simulink model "Main_SpeedOptimisedVersionTannenweg"  (R2024b)
settings: Solver=ode15s  StartTime=0.0  StopTime=3600*2  FixedStep=0.1  RelTol=0.001
model workspace (MAT data in the model file):
  Ti = 5
  fa = 0.00071
  fd = 0.03
  ips = 36
  ma = 0.0013
  md = 0.04
  roomarea1 = 20
  s = 15
libraries: fl_lib x1434, nesl_utility x105, SimscapeFluids_lib x35
(part 4 of 22)

== system Main_SpeedOptimisedVersionTannenweg/EG/Raum12 ==
  Tatm : Inport
  valve command : Inport  Port=2
  Air-InnerDoor Convection1 : fl_lib/Thermal/Thermal Elements/Convective Heat Transfer  thermal_type=foundation.enum.constant_variable.constant  area=1.8 m^2  heat_tr_coeff=8 W/m^2/K  min_heat_tr_coeff=1e-3 W/(K*m^2)  T_specify=off  T_priority=High  T=0 K  T_nominal_specify=off  T_nominal_value=1  T_nominal_unit=K  Q_specify=off  Q_priority=High  Q=0 J/s  Q_nominal_specify=off  Q_nominal_value=1  Q_nominal_unit=W
  Controlled Temperature Source : fl_lib/Thermal/Thermal Sources/Controlled Temperature Source
  Flur12OG2 : fl_lib/Thermal/Thermal Elements/Convective Heat Transfer  thermal_type=foundation.enum.constant_variable.constant  area=19.68 m^2  heat_tr_coeff=8 W/m^2/K  min_heat_tr_coeff=1e-3 W/(K*m^2)  T_specify=off  T_priority=High  T=0 K  T_nominal_specify=off  T_nominal_value=1  T_nominal_unit=K  Q_specify=off  Q_priority=High  Q=0 J/s  Q_nominal_specify=off  Q_nominal_value=1  Q_nominal_unit=W
  Half Flur12OG2 : fl_lib/Thermal/Thermal Elements/Conductive Heat Transfer  thermal_type=foundation.enum.ConstantVariableTabulated.Constant  wall_geometry=foundation.enum.ConductionWallGeometry.Planar  area=19.68 m^2  thickness=.15 m  d_in=0.05 m  d_out=0.1 m  L=1 m  th_cond_min=10 W/(K*m)  th_cond=.32 W/m/K  th_cond_TLU=[413, 401, 392, 383, 371, 357, 342] W/(K*m)  temp_TLU=[200, 273, 400, 600, 800, 1000, 1200] K  T_specify=off  T_priority=High  T=0 K  T_nominal_specify=off  T_nominal_value=1  T_nominal_unit=K  Q_specify=off  Q_priority=High  Q=0 J/s  Q_nominal_specify=off  Q_nominal_value=1  Q_nominal_unit=W
  Half IW1-Air4 : fl_lib/Thermal/Thermal Elements/Conductive Heat Transfer  thermal_type=foundation.enum.ConstantVariableTabulated.Constant  wall_geometry=foundation.enum.ConductionWallGeometry.Planar  area=3.1 m^2  thickness=.16 m  d_in=0.05 m  d_out=0.1 m  L=1 m  th_cond_min=10 W/(K*m)  th_cond=.069 W/m/K  th_cond_TLU=[413, 401, 392, 383, 371, 357, 342] W/(K*m)  temp_TLU=[200, 273, 400, 600, 800, 1000, 1200] K  T_specify=off  T_priority=High  T=0 K  T_nominal_specify=off  T_nominal_value=1  T_nominal_unit=K  Q_specify=off  Q_priority=High  Q=0 J/s  Q_nominal_specify=off  Q_nominal_value=1  Q_nominal_unit=W
  Half Wall-Air Conduction1 : fl_lib/Thermal/Thermal Elements/Conductive Heat Transfer  thermal_type=foundation.enum.ConstantVariableTabulated.Constant  wall_geometry=foundation.enum.ConductionWallGeometry.Planar  area=3.7 m^2  thickness=.16 m  d_in=0.05 m  d_out=0.1 m  L=1 m  th_cond_min=10 W/(K*m)  th_cond=.069 W/m/K  th_cond_TLU=[413, 401, 392, 383, 371, 357, 342] W/(K*m)  temp_TLU=[200, 273, 400, 600, 800, 1000, 1200] K  T_specify=off  T_priority=High  T=0 K  T_nominal_specify=off  T_nominal_value=1  T_nominal_unit=K  Q_specify=off  Q_priority=High  Q=0 J/s  Q_nominal_specify=off  Q_nominal_value=1  Q_nominal_unit=W
  Half Wall-Air Conduction2 : fl_lib/Thermal/Thermal Elements/Conductive Heat Transfer  thermal_type=foundation.enum.ConstantVariableTabulated.Constant  wall_geometry=foundation.enum.ConductionWallGeometry.Planar  area=8.4 m^2  thickness=.16 m  d_in=0.05 m  d_out=0.1 m  L=1 m  th_cond_min=10 W/(K*m)  th_cond=.069 W/m/K  th_cond_TLU=[413, 401, 392, 383, 371, 357, 342] W/(K*m)  temp_TLU=[200, 273, 400, 600, 800, 1000, 1200] K  T_specify=off  T_priority=High  T=0 K  T_nominal_specify=off  T_nominal_value=1  T_nominal_unit=K  Q_specify=off  Q_priority=High  Q=0 J/s  Q_nominal_specify=off  Q_nominal_value=1  Q_nominal_unit=W
  Half Wall-Air Conduction3 : fl_lib/Thermal/Thermal Elements/Conductive Heat Transfer  thermal_type=foundation.enum.ConstantVariableTabulated.Constant  wall_geometry=foundation.enum.ConductionWallGeometry.Planar  area=12.5 m^2  thickness=.16 m  d_in=0.05 m  d_out=0.1 m  L=1 m  th_cond_min=10 W/(K*m)  th_cond=.069 W/m/K  th_cond_TLU=[413, 401, 392, 383, 371, 357, 342] W/(K*m)  temp_TLU=[200, 273, 400, 600, 800, 1000, 1200] K  T_specify=off  T_priority=High  T=0 K  T_nominal_specify=off  T_nominal_value=1  T_nominal_unit=K  Q_specify=off  Q_priority=High  Q=0 J/s  Q_nominal_specify=off  Q_nominal_value=1  Q_nominal_unit=W
  Half Window-Air Conduction1 : fl_lib/Thermal/Thermal Elements/Conductive Heat Transfer  thermal_type=foundation.enum.ConstantVariableTabulated.Constant  wall_geometry=foundation.enum.ConductionWallGeometry.Planar  area=1.8 m^2  thickness=.022 m  d_in=0.05 m  d_out=0.1 m  L=1 m  th_cond_min=10 W/(K*m)  th_cond=.13 W/m/K  th_cond_TLU=[413, 401, 392, 383, 371, 357, 342] W/(K*m)  temp_TLU=[200, 273, 400, 600, 800, 1000, 1200] K  T_specify=off  T_priority=High  T=0 K  T_nominal_specify=off  T_nominal_value=1  T_nominal_unit=K  Q_specify=off  Q_priority=High  Q=0 J/s  Q_nominal_specify=off  Q_nominal_value=1  Q_nominal_unit=W
  Heater : Subsystem
      settings: PortSchema="{\"entries\":[{\"content\":{\"sides\":[{\"content\":{\"connectorIds\":[\"In1\"]},\"type\":\"ConnectorPlacement.EquallySpacedRectSide\",\"uuid\":\"7b4379d5-fe86-4f5f-b347-17463247d5cb\"},{\"content\":{\"connectorIds\":[\"RConn1\"],\"side\":\"RIGHT\"},\"type\":\"ConnectorPlacement.EquallySpacedRectSide\",\"uuid\":\"add3919f-9a79-4726-aacf-5344366c736f\"},{\"content\":{\"connectorIds\":[\"LConn1\"],\"side\":\"TOP\"},\"type\":\"ConnectorPlacement.EquallySpacedRectSide\",\"uuid\":\"2be7b118-9114-410d-904a-4756a3068fbb\"},{\"content\":{\"connectorIds\":[\"RConn2\"],\"side\":\"BOTTOM\"},\"type\":\"ConnectorPlacement.EquallySpacedRectSide\",\"uuid\":\"3477f1e1-5c09-4719-a7a1-17d4fd79a7ad\"}]},\"type\":\"ConnectorPlacement.EquallySpacedConnector\",\"uuid\":\"01d92670-8519-469a-8463-0c3952b88216\"}],\"packageUris\":[\"http://schema.mathworks.com/mf0/Connector/R2020b\"],\"version\":\"1.0\"}"
  IW12-11 : fl_lib/Thermal/Thermal Elements/Convective Heat Transfer  thermal_type=foundation.enum.constant_variable.constant  area=12.5 m^2  heat_tr_coeff=8 W/m^2/K  min_heat_tr_coeff=1e-3 W/(K*m^2)  T_specify=off  T_priority=High  T=0 K  T_nominal_specify=off  T_nominal_value=1  T_nominal_unit=K  Q_specify=off  Q_priority=High  Q=0 J/s  Q_nominal_specify=off  Q_nominal_value=1  Q_nominal_unit=W
  IW12-2 : fl_lib/Thermal/Thermal Elements/Convective Heat Transfer  thermal_type=foundation.enum.constant_variable.constant  area=3.7 m^2  heat_tr_coeff=8 W/m^2/K  min_heat_tr_coeff=1e-3 W/(K*m^2)  T_specify=off  T_priority=High  T=0 K  T_nominal_specify=off  T_nominal_value=1  T_nominal_unit=K  Q_specify=off  Q_priority=High  Q=0 J/s  Q_nominal_specify=off  Q_nominal_value=1  Q_nominal_unit=W
  IW12-3 : fl_lib/Thermal/Thermal Elements/Convective Heat Transfer  thermal_type=foundation.enum.constant_variable.constant  area=8.4 m^2  heat_tr_coeff=8 W/m^2/K  min_heat_tr_coeff=1e-3 W/(K*m^2)  T_specify=off  T_priority=High  T=0 K  T_nominal_specify=off  T_nominal_value=1  T_nominal_unit=K  Q_specify=off  Q_priority=High  Q=0 J/s  Q_nominal_specify=off  Q_nominal_value=1  Q_nominal_unit=W
  IW5 : fl_lib/Thermal/Thermal Elements/Convective Heat Transfer  thermal_type=foundation.enum.constant_variable.constant  area=3.1 m^2  heat_tr_coeff=8 W/m^2/K  min_heat_tr_coeff=1e-3 W/(K*m^2)  T_specify=off  T_priority=High  T=0 K  T_nominal_specify=off  T_nominal_value=1  T_nominal_unit=K  Q_specify=off  Q_priority=High  Q=0 J/s  Q_nominal_specify=off  Q_nominal_value=1  Q_nominal_unit=W
  Simulink-PS Converter3 : nesl_utility/Simulink-PS Converter  PhysicalDomain=network_engine_domain  SubClassName=ps_input  LeftPortType=input  RightPortType=output  PseudoPeriodic=off  Frequencies=[]  NoiseDistribution=none  NoiseParameters=[]  Unit=degC  AffineConversion=on  FilteringAndDerivatives=zero  SimscapeFilterOrder=1  InputFilterTimeConstant=.001  UdotUserProvided=0
  Temp. Sensor : Subsystem
  Thermal Mass Air : fl_lib/Thermal/Thermal Elements/Thermal Mass  mass_type=foundation.enum.constant_variable.constant  mass=60.4 kg  sp_heat=1005 J/kg/K  mass_min=1e-6 kg  num_ports=foundation.enum.numPorts2.one  m_specify=off  m_priority=High  m=1 kg  m_nominal_specify=off  m_nominal_value=1  m_nominal_unit=kg  T_specify=on  T_priority=High  T=Ti degC  T_nominal_specify=off  T_nominal_value=1  T_nominal_unit=K  Q_specify=off  Q_priority=None  Q=0 W  Q_nominal_specify=off  Q_nominal_value=1  Q_nominal_unit=W
  Thermal Mass Flur12OG2 : fl_lib/Thermal/Thermal Elements/Thermal Mass  mass_type=foundation.enum.constant_variable.constant  mass=5547 kg  sp_heat=889 J/kg/K  mass_min=1e-6 kg  num_ports=foundation.enum.numPorts2.one  m_specify=off  m_priority=High  m=1 kg  m_nominal_specify=off  m_nominal_value=1  m_nominal_unit=kg  T_specify=on  T_priority=High  T=Ti degC  T_nominal_specify=off  T_nominal_value=1  T_nominal_unit=K  Q_specify=off  Q_priority=None  Q=0 W  Q_nominal_specify=off  Q_nominal_value=1  Q_nominal_unit=W
  Thermal Mass IW1 : fl_lib/Thermal/Thermal Elements/Thermal Mass  mass_type=foundation.enum.constant_variable.constant  mass=8.4*547*.3*.5 kg  sp_heat=876 J/kg/K  mass_min=1e-6 kg  num_ports=foundation.enum.numPorts2.one  m_specify=off  m_priority=High  m=1 kg  m_nominal_specify=off  m_nominal_value=1  m_nominal_unit=kg  T_specify=on  T_priority=High  T=Ti degC  T_nominal_specify=off  T_nominal_value=1  T_nominal_unit=K  Q_specify=off  Q_priority=None  Q=0 W  Q_nominal_specify=off  Q_nominal_value=1  Q_nominal_unit=W
  Thermal Mass IW12 : fl_lib/Thermal/Thermal Elements/Thermal Mass  mass_type=foundation.enum.constant_variable.constant  mass=3.7*547*.3*.5 kg  sp_heat=876 J/kg/K  mass_min=1e-6 kg  num_ports=foundation.enum.numPorts2.one  m_specify=off  m_priority=High  m=1 kg  m_nominal_specify=off  m_nominal_value=1  m_nominal_unit=kg  T_specify=on  T_priority=High  T=Ti degC  T_nominal_specify=off  T_nominal_value=1  T_nominal_unit=K  Q_specify=off  Q_priority=None  Q=0 W  Q_nominal_specify=off  Q_nominal_value=1  Q_nominal_unit=W
  Thermal Mass IW2 : fl_lib/Thermal/Thermal Elements/Thermal Mass  mass_type=foundation.enum.constant_variable.constant  mass=12.5*547*.3*.5 kg  sp_heat=876 J/kg/K  mass_min=1e-6 kg  num_ports=foundation.enum.numPorts2.one  m_specify=off  m_priority=High  m=1 kg  m_nominal_specify=off  m_nominal_value=1  m_nominal_unit=kg  T_specify=on  T_priority=High  T=Ti degC  T_nominal_specify=off  T_nominal_value=1  T_nominal_unit=K  Q_specify=off  Q_priority=None  Q=0 W  Q_nominal_specify=off  Q_nominal_value=1  Q_nominal_unit=W
  Thermal Mass IW5 : fl_lib/Thermal/Thermal Elements/Thermal Mass  mass_type=foundation.enum.constant_variable.constant  mass=1 kg  sp_heat=1600 J/kg/K  mass_min=1e-6 kg  num_ports=foundation.enum.numPorts2.one  m_specify=off  m_priority=High  m=1 kg  m_nominal_specify=off  m_nominal_value=1  m_nominal_unit=kg  T_specify=on  T_priority=High  T=Ti degC  T_nominal_specify=off  T_nominal_value=1  T_nominal_unit=K  Q_specify=off  Q_priority=None  Q=0 W  Q_nominal_specify=off  Q_nominal_value=1  Q_nominal_unit=W
  Thermal Mass InnerDoor : fl_lib/Thermal/Thermal Elements/Thermal Mass  mass_type=foundation.enum.constant_variable.constant  mass=36 kg  sp_heat=1600 J/kg/K  mass_min=1e-6 kg  num_ports=foundation.enum.numPorts2.one  m_specify=off  m_priority=High  m=1 kg  m_nominal_specify=off  m_nominal_value=1  m_nominal_unit=kg  T_specify=on  T_priority=High  T=Ti degC  T_nominal_specify=off  T_nominal_value=1  T_nominal_unit=K  Q_specify=off  Q_priority=None  Q=0 W  Q_nominal_specify=off  Q_nominal_value=1  Q_nominal_unit=W
  Thermal Reference1 : fl_lib/Thermal/Thermal Elements/Thermal Reference
  X-Atm : Subsystem
  Hot Water In1 : PMIOPort  Side=Left
  Hot Water Out1 : PMIOPort  Port=2  Side=Left
  Y-6 Flur12OG2 : PMIOPort  Port=3  Side=Left
  12-11 : PMIOPort  Port=4  Side=Right
  Door12 : PMIOPort  Port=5  Side=Right
  12-3 : PMIOPort  Port=6  Side=Right
  12-2 : PMIOPort  Port=7  Side=Right
  Troom : Outport
  wires:
  Tatm/1 -> Simulink-PS Converter3/1
  Temp. Sensor/1(T) -> Troom/1
  valve command/1 -> Heater/1(valve command)
  connections:
  Flur12OG2/RConn1 -- Half Flur12OG2/LConn1
  Half Flur12OG2/RConn1 -- Thermal Mass Flur12OG2/LConn1 -- Y-6 Flur12OG2/RConn1
  IW5/RConn1 -- Half IW1-Air4/LConn1
  Thermal Mass IW5/LConn1 -- Half IW1-Air4/RConn1
  Heater/RConn2 -- Hot Water Out1/RConn1
  Hot Water In1/RConn1 -- Heater/LConn1
  X-Atm/RConn1 -- Controlled Temperature Source/LConn1
  IW12-11/LConn1 -- Flur12OG2/LConn1 -- IW5/LConn1 -- Air-InnerDoor Convection1/LConn1 -- IW12-3/LConn1 -- Heater/RConn1 -- Thermal Mass Air/LConn1 -- X-Atm/LConn1 -- Temp. Sensor/LConn1 -- IW12-2/LConn1
  Controlled Temperature Source/RConn1 -- Simulink-PS Converter3/RConn1
  Thermal Reference1/LConn1 -- Controlled Temperature Source/RConn2
  12-3/RConn1 -- Thermal Mass IW1/LConn1 -- Half Wall-Air Conduction2/RConn1
  Thermal Mass InnerDoor/LConn1 -- Half Window-Air Conduction1/RConn1 -- Door12/RConn1
  Half Wall-Air Conduction3/RConn1 -- Thermal Mass IW2/LConn1 -- 12-11/RConn1
  12-2/RConn1 -- Half Wall-Air Conduction1/RConn1 -- Thermal Mass IW12/LConn1
  IW12-11/RConn1 -- Half Wall-Air Conduction3/LConn1
  Air-InnerDoor Convection1/RConn1 -- Half Window-Air Conduction1/LConn1
  IW12-2/RConn1 -- Half Wall-Air Conduction1/LConn1
  IW12-3/RConn1 -- Half Wall-Air Conduction2/LConn1

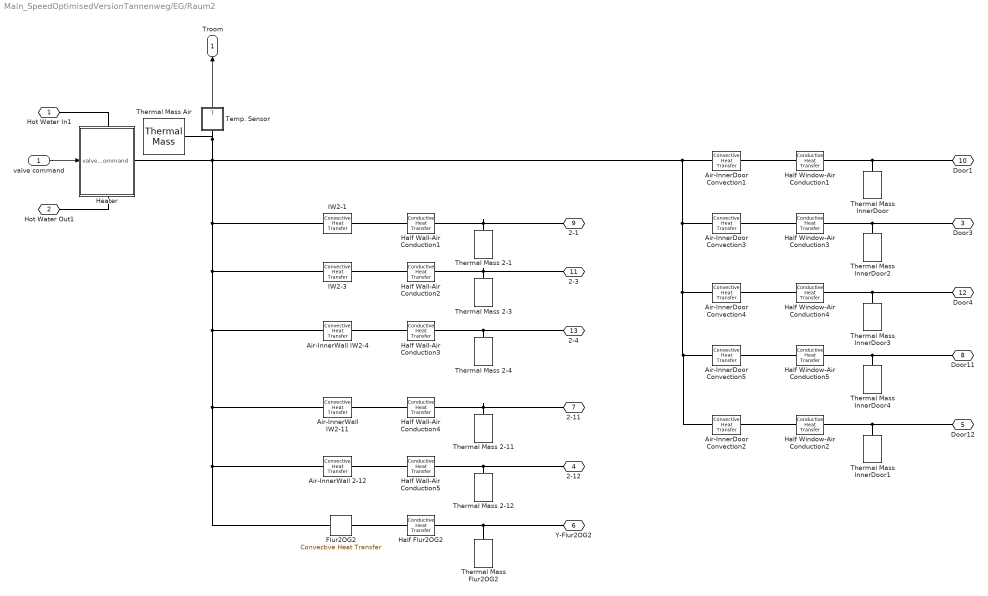
== system Main_SpeedOptimisedVersionTannenweg/EG/Raum2 ==
  valve command : Inport
  Air-InnerDoor Convection{1..5} (5 alike) : fl_lib/Thermal/Thermal Elements/Convective Heat Transfer  thermal_type=foundation.enum.constant_variable.constant  area=8.4 m^2  heat_tr_coeff=8 W/m^2/K  min_heat_tr_coeff=1e-3 W/(K*m^2)  T_specify=off  T_priority=High  T=0 K  T_nominal_specify=off  T_nominal_value=1  T_nominal_unit=K  Q_specify=off  Q_priority=High  Q=0 J/s  Q_nominal_specify=off  Q_nominal_value=1  Q_nominal_unit=W
  Air-InnerWall 2-12 : fl_lib/Thermal/Thermal Elements/Convective Heat Transfer  thermal_type=foundation.enum.constant_variable.constant  area=3.7 m^2  heat_tr_coeff=8 W/m^2/K  min_heat_tr_coeff=1e-3 W/(K*m^2)  T_specify=off  T_priority=High  T=0 K  T_nominal_specify=off  T_nominal_value=1  T_nominal_unit=K  Q_specify=off  Q_priority=High  Q=0 J/s  Q_nominal_specify=off  Q_nominal_value=1  Q_nominal_unit=W
  Air-InnerWall IW2-11 : fl_lib/Thermal/Thermal Elements/Convective Heat Transfer  thermal_type=foundation.enum.constant_variable.constant  area=1.8 m^2  heat_tr_coeff=8 W/m^2/K  min_heat_tr_coeff=1e-3 W/(K*m^2)  T_specify=off  T_priority=High  T=0 K  T_nominal_specify=off  T_nominal_value=1  T_nominal_unit=K  Q_specify=off  Q_priority=High  Q=0 J/s  Q_nominal_specify=off  Q_nominal_value=1  Q_nominal_unit=W
  Air-InnerWall IW2-4 : fl_lib/Thermal/Thermal Elements/Convective Heat Transfer  thermal_type=foundation.enum.constant_variable.constant  area=5.2 m^2  heat_tr_coeff=8 W/m^2/K  min_heat_tr_coeff=1e-3 W/(K*m^2)  T_specify=off  T_priority=High  T=0 K  T_nominal_specify=off  T_nominal_value=1  T_nominal_unit=K  Q_specify=off  Q_priority=High  Q=0 J/s  Q_nominal_specify=off  Q_nominal_value=1  Q_nominal_unit=W
  Flur2OG2 : fl_lib/Thermal/Thermal Elements/Convective Heat Transfer  thermal_type=foundation.enum.constant_variable.constant  area=5.33 m^2  heat_tr_coeff=8 W/m^2/K  min_heat_tr_coeff=1e-3 W/(K*m^2)  T_specify=off  T_priority=High  T=0 K  T_nominal_specify=off  T_nominal_value=1  T_nominal_unit=K  Q_specify=off  Q_priority=High  Q=0 J/s  Q_nominal_specify=off  Q_nominal_value=1  Q_nominal_unit=W
  Half Flur2OG2 : fl_lib/Thermal/Thermal Elements/Conductive Heat Transfer  thermal_type=foundation.enum.ConstantVariableTabulated.Constant  wall_geometry=foundation.enum.ConductionWallGeometry.Planar  area=5.33 m^2  thickness=.15 m  d_in=0.05 m  d_out=0.1 m  L=1 m  th_cond_min=10 W/(K*m)  th_cond=.32 W/m/K  th_cond_TLU=[413, 401, 392, 383, 371, 357, 342] W/(K*m)  temp_TLU=[200, 273, 400, 600, 800, 1000, 1200] K  T_specify=off  T_priority=High  T=0 K  T_nominal_specify=off  T_nominal_value=1  T_nominal_unit=K  Q_specify=off  Q_priority=High  Q=0 J/s  Q_nominal_specify=off  Q_nominal_value=1  Q_nominal_unit=W
  Half Wall-Air Conduction1 : fl_lib/Thermal/Thermal Elements/Conductive Heat Transfer  thermal_type=foundation.enum.ConstantVariableTabulated.Constant  wall_geometry=foundation.enum.ConductionWallGeometry.Planar  area=3.8 m^2  thickness=.16 m  d_in=0.05 m  d_out=0.1 m  L=1 m  th_cond_min=10 W/(K*m)  th_cond=.069 W/m/K  th_cond_TLU=[413, 401, 392, 383, 371, 357, 342] W/(K*m)  temp_TLU=[200, 273, 400, 600, 800, 1000, 1200] K  T_specify=off  T_priority=High  T=0 K  T_nominal_specify=off  T_nominal_value=1  T_nominal_unit=K  Q_specify=off  Q_priority=High  Q=0 J/s  Q_nominal_specify=off  Q_nominal_value=1  Q_nominal_unit=W
  Half Wall-Air Conduction2 : fl_lib/Thermal/Thermal Elements/Conductive Heat Transfer  thermal_type=foundation.enum.ConstantVariableTabulated.Constant  wall_geometry=foundation.enum.ConductionWallGeometry.Planar  area=6.7 m^2  thickness=.16 m  d_in=0.05 m  d_out=0.1 m  L=1 m  th_cond_min=10 W/(K*m)  th_cond=.069 W/m/K  th_cond_TLU=[413, 401, 392, 383, 371, 357, 342] W/(K*m)  temp_TLU=[200, 273, 400, 600, 800, 1000, 1200] K  T_specify=off  T_priority=High  T=0 K  T_nominal_specify=off  T_nominal_value=1  T_nominal_unit=K  Q_specify=off  Q_priority=High  Q=0 J/s  Q_nominal_specify=off  Q_nominal_value=1  Q_nominal_unit=W
  Half Wall-Air Conduction3 : fl_lib/Thermal/Thermal Elements/Conductive Heat Transfer  thermal_type=foundation.enum.ConstantVariableTabulated.Constant  wall_geometry=foundation.enum.ConductionWallGeometry.Planar  area=5.2 m^2  thickness=.16 m  d_in=0.05 m  d_out=0.1 m  L=1 m  th_cond_min=10 W/(K*m)  th_cond=.069 W/m/K  th_cond_TLU=[413, 401, 392, 383, 371, 357, 342] W/(K*m)  temp_TLU=[200, 273, 400, 600, 800, 1000, 1200] K  T_specify=off  T_priority=High  T=0 K  T_nominal_specify=off  T_nominal_value=1  T_nominal_unit=K  Q_specify=off  Q_priority=High  Q=0 J/s  Q_nominal_specify=off  Q_nominal_value=1  Q_nominal_unit=W
  Half Wall-Air Conduction4 : fl_lib/Thermal/Thermal Elements/Conductive Heat Transfer  thermal_type=foundation.enum.ConstantVariableTabulated.Constant  wall_geometry=foundation.enum.ConductionWallGeometry.Planar  area=1.8 m^2  thickness=.16 m  d_in=0.05 m  d_out=0.1 m  L=1 m  th_cond_min=10 W/(K*m)  th_cond=.069 W/m/K  th_cond_TLU=[413, 401, 392, 383, 371, 357, 342] W/(K*m)  temp_TLU=[200, 273, 400, 600, 800, 1000, 1200] K  T_specify=off  T_priority=High  T=0 K  T_nominal_specify=off  T_nominal_value=1  T_nominal_unit=K  Q_specify=off  Q_priority=High  Q=0 J/s  Q_nominal_specify=off  Q_nominal_value=1  Q_nominal_unit=W
  Half Wall-Air Conduction5 : fl_lib/Thermal/Thermal Elements/Conductive Heat Transfer  thermal_type=foundation.enum.ConstantVariableTabulated.Constant  wall_geometry=foundation.enum.ConductionWallGeometry.Planar  area=3.7 m^2  thickness=.16 m  d_in=0.05 m  d_out=0.1 m  L=1 m  th_cond_min=10 W/(K*m)  th_cond=.069 W/m/K  th_cond_TLU=[413, 401, 392, 383, 371, 357, 342] W/(K*m)  temp_TLU=[200, 273, 400, 600, 800, 1000, 1200] K  T_specify=off  T_priority=High  T=0 K  T_nominal_specify=off  T_nominal_value=1  T_nominal_unit=K  Q_specify=off  Q_priority=High  Q=0 J/s  Q_nominal_specify=off  Q_nominal_value=1  Q_nominal_unit=W
  Half Window-Air Conduction{1..5} (5 alike) : fl_lib/Thermal/Thermal Elements/Conductive Heat Transfer  thermal_type=foundation.enum.ConstantVariableTabulated.Constant  wall_geometry=foundation.enum.ConductionWallGeometry.Planar  area=8.4 m^2  thickness=.022 m  d_in=0.05 m  d_out=0.1 m  L=1 m  th_cond_min=10 W/(K*m)  th_cond=.13 W/m/K  th_cond_TLU=[413, 401, 392, 383, 371, 357, 342] W/(K*m)  temp_TLU=[200, 273, 400, 600, 800, 1000, 1200] K  T_specify=off  T_priority=High  T=0 K  T_nominal_specify=off  T_nominal_value=1  T_nominal_unit=K  Q_specify=off  Q_priority=High  Q=0 J/s  Q_nominal_specify=off  Q_nominal_value=1  Q_nominal_unit=W
  Heater : Subsystem
      settings: PortSchema="{\"entries\":[{\"content\":{\"sides\":[{\"content\":{\"connectorIds\":[\"In1\"]},\"type\":\"ConnectorPlacement.EquallySpacedRectSide\",\"uuid\":\"7b4379d5-fe86-4f5f-b347-17463247d5cb\"},{\"content\":{\"connectorIds\":[\"RConn1\"],\"side\":\"RIGHT\"},\"type\":\"ConnectorPlacement.EquallySpacedRectSide\",\"uuid\":\"add3919f-9a79-4726-aacf-5344366c736f\"},{\"content\":{\"connectorIds\":[\"LConn1\"],\"side\":\"TOP\"},\"type\":\"ConnectorPlacement.EquallySpacedRectSide\",\"uuid\":\"2be7b118-9114-410d-904a-4756a3068fbb\"},{\"content\":{\"connectorIds\":[\"RConn2\"],\"side\":\"BOTTOM\"},\"type\":\"ConnectorPlacement.EquallySpacedRectSide\",\"uuid\":\"3477f1e1-5c09-4719-a7a1-17d4fd79a7ad\"}]},\"type\":\"ConnectorPlacement.EquallySpacedConnector\",\"uuid\":\"01d92670-8519-469a-8463-0c3952b88216\"}],\"packageUris\":[\"http://schema.mathworks.com/mf0/Connector/R2020b\"],\"version\":\"1.0\"}"
  IW2-1 : fl_lib/Thermal/Thermal Elements/Convective Heat Transfer  thermal_type=foundation.enum.constant_variable.constant  area=3.8 m^2  heat_tr_coeff=8 W/m^2/K  min_heat_tr_coeff=1e-3 W/(K*m^2)  T_specify=off  T_priority=High  T=0 K  T_nominal_specify=off  T_nominal_value=1  T_nominal_unit=K  Q_specify=off  Q_priority=High  Q=0 J/s  Q_nominal_specify=off  Q_nominal_value=1  Q_nominal_unit=W
  IW2-3 : fl_lib/Thermal/Thermal Elements/Convective Heat Transfer  thermal_type=foundation.enum.constant_variable.constant  area=6.7 m^2  heat_tr_coeff=8 W/m^2/K  min_heat_tr_coeff=1e-3 W/(K*m^2)  T_specify=off  T_priority=High  T=0 K  T_nominal_specify=off  T_nominal_value=1  T_nominal_unit=K  Q_specify=off  Q_priority=High  Q=0 J/s  Q_nominal_specify=off  Q_nominal_value=1  Q_nominal_unit=W
  Temp. Sensor : Subsystem
  Thermal Mass 2-1 : fl_lib/Thermal/Thermal Elements/Thermal Mass  mass_type=foundation.enum.constant_variable.constant  mass=547*.5*.3*3.8 kg  sp_heat=876 J/kg/K  mass_min=1e-6 kg  num_ports=foundation.enum.numPorts2.one  m_specify=off  m_priority=High  m=1 kg  m_nominal_specify=off  m_nominal_value=1  m_nominal_unit=kg  T_specify=on  T_priority=High  T=Ti degC  T_nominal_specify=off  T_nominal_value=1  T_nominal_unit=K  Q_specify=off  Q_priority=None  Q=0 W  Q_nominal_specify=off  Q_nominal_value=1  Q_nominal_unit=W
  Thermal Mass 2-11 : fl_lib/Thermal/Thermal Elements/Thermal Mass  mass_type=foundation.enum.constant_variable.constant  mass=1.8*547*.15 kg  sp_heat=876 J/kg/K  mass_min=1e-6 kg  num_ports=foundation.enum.numPorts2.one  m_specify=off  m_priority=High  m=1 kg  m_nominal_specify=off  m_nominal_value=1  m_nominal_unit=kg  T_specify=on  T_priority=High  T=Ti degC  T_nominal_specify=off  T_nominal_value=1  T_nominal_unit=K  Q_specify=off  Q_priority=None  Q=0 W  Q_nominal_specify=off  Q_nominal_value=1  Q_nominal_unit=W
  Thermal Mass 2-12 : fl_lib/Thermal/Thermal Elements/Thermal Mass  mass_type=foundation.enum.constant_variable.constant  mass=3.7*547*.15 kg  sp_heat=876 J/kg/K  mass_min=1e-6 kg  num_ports=foundation.enum.numPorts2.one  m_specify=off  m_priority=High  m=1 kg  m_nominal_specify=off  m_nominal_value=1  m_nominal_unit=kg  T_specify=on  T_priority=High  T=Ti degC  T_nominal_specify=off  T_nominal_value=1  T_nominal_unit=K  Q_specify=off  Q_priority=None  Q=0 W  Q_nominal_specify=off  Q_nominal_value=1  Q_nominal_unit=W
  Thermal Mass 2-3 : fl_lib/Thermal/Thermal Elements/Thermal Mass  mass_type=foundation.enum.constant_variable.constant  mass=6.7*.15*547 kg  sp_heat=876 J/kg/K  mass_min=1e-6 kg  num_ports=foundation.enum.numPorts2.one  m_specify=off  m_priority=High  m=1 kg  m_nominal_specify=off  m_nominal_value=1  m_nominal_unit=kg  T_specify=on  T_priority=High  T=Ti degC  T_nominal_specify=off  T_nominal_value=1  T_nominal_unit=K  Q_specify=off  Q_priority=None  Q=0 W  Q_nominal_specify=off  Q_nominal_value=1  Q_nominal_unit=W
  Thermal Mass 2-4 : fl_lib/Thermal/Thermal Elements/Thermal Mass  mass_type=foundation.enum.constant_variable.constant  mass=547*.15*5.2 kg  sp_heat=876 J/kg/K  mass_min=1e-6 kg  num_ports=foundation.enum.numPorts2.one  m_specify=off  m_priority=High  m=1 kg  m_nominal_specify=off  m_nominal_value=1  m_nominal_unit=kg  T_specify=on  T_priority=High  T=Ti degC  T_nominal_specify=off  T_nominal_value=1  T_nominal_unit=K  Q_specify=off  Q_priority=None  Q=0 W  Q_nominal_specify=off  Q_nominal_value=1  Q_nominal_unit=W
  Thermal Mass Air : fl_lib/Thermal/Thermal Elements/Thermal Mass  mass_type=foundation.enum.constant_variable.constant  mass=16.4 kg  sp_heat=1005 J/kg/K  mass_min=1e-6 kg  num_ports=foundation.enum.numPorts2.one  m_specify=off  m_priority=High  m=1 kg  m_nominal_specify=off  m_nominal_value=1  m_nominal_unit=kg  T_specify=on  T_priority=High  T=Ti degC  T_nominal_specify=off  T_nominal_value=1  T_nominal_unit=K  Q_specify=off  Q_priority=None  Q=0 W  Q_nominal_specify=off  Q_nominal_value=1  Q_nominal_unit=W
  Thermal Mass Flur2OG2 : fl_lib/Thermal/Thermal Elements/Thermal Mass  mass_type=foundation.enum.constant_variable.constant  mass=1502 kg  sp_heat=889 J/kg/K  mass_min=1e-6 kg  num_ports=foundation.enum.numPorts2.one  m_specify=off  m_priority=High  m=1 kg  m_nominal_specify=off  m_nominal_value=1  m_nominal_unit=kg  T_specify=on  T_priority=High  T=Ti degC  T_nominal_specify=off  T_nominal_value=1  T_nominal_unit=K  Q_specify=off  Q_priority=None  Q=0 W  Q_nominal_specify=off  Q_nominal_value=1  Q_nominal_unit=W
  Thermal Mass InnerDoor{,1..4} (5 alike) : fl_lib/Thermal/Thermal Elements/Thermal Mass  mass_type=foundation.enum.constant_variable.constant  mass=170 kg  sp_heat=1600 J/kg/K  mass_min=1e-6 kg  num_ports=foundation.enum.numPorts2.one  m_specify=off  m_priority=High  m=1 kg  m_nominal_specify=off  m_nominal_value=1  m_nominal_unit=kg  T_specify=on  T_priority=High  T=Ti degC  T_nominal_specify=off  T_nominal_value=1  T_nominal_unit=K  Q_specify=off  Q_priority=None  Q=0 W  Q_nominal_specify=off  Q_nominal_value=1  Q_nominal_unit=W
  Hot Water In1 : PMIOPort  Side=Left
  Hot Water Out1 : PMIOPort  Port=2  Side=Left
  Door3 : PMIOPort  Port=3  Side=Left
  2-12 : PMIOPort  Port=4  Side=Left
  Door12 : PMIOPort  Port=5  Side=Left
  Y-Flur2OG2 : PMIOPort  Port=6  Side=Left
  2-11 : PMIOPort  Port=7  Side=Right
  Door11 : PMIOPort  Port=8  Side=Right
  2-1 : PMIOPort  Port=9  Side=Right
  Door1 : PMIOPort  Port=10  Side=Right
  2-3 : PMIOPort  Port=11  Side=Right
  Door4 : PMIOPort  Port=12  Side=Right
  2-4 : PMIOPort  Port=13  Side=Right
  Troom : Outport
  wires:
  Temp. Sensor/1(T) -> Troom/1
  valve command/1 -> Heater/1(valve command)
  connections:
  Heater/RConn2 -- Hot Water Out1/RConn1
  Hot Water In1/RConn1 -- Heater/LConn1
  Air-InnerWall IW2-11/LConn1 -- IW2-3/LConn1 -- IW2-1/LConn1 -- Air-InnerDoor Convection5/LConn1 -- Air-InnerDoor Convection2/LConn1 -- Air-InnerDoor Convection4/LConn1 -- Air-InnerDoor Convection3/LConn1 -- Air-InnerDoor Convection1/LConn1 -- Heater/RConn1 -- Thermal Mass Air/LConn1 -- Temp. Sensor/LConn1 -- Air-InnerWall IW2-4/LConn1 -- Flur2OG2/LConn1 -- Air-InnerWall 2-12/LConn1
  Half Window-Air Conduction3/RConn1 -- Door3/RConn1 -- Thermal Mass InnerDoor2/LConn1
  Thermal Mass 2-1/LConn1 -- Half Wall-Air Conduction1/RConn1 -- 2-1/RConn1
  Thermal Mass 2-3/LConn1 -- 2-3/RConn1 -- Half Wall-Air Conduction2/RConn1
  Thermal Mass InnerDoor3/LConn1 -- Door4/RConn1 -- Half Window-Air Conduction4/RConn1
  Thermal Mass 2-11/LConn1 -- 2-11/RConn1 -- Half Wall-Air Conduction4/RConn1
  Half Window-Air Conduction5/RConn1 -- Door11/RConn1 -- Thermal Mass InnerDoor4/LConn1
  Half Wall-Air Conduction5/RConn1 -- 2-12/RConn1 -- Thermal Mass 2-12/LConn1
  Thermal Mass InnerDoor/LConn1 -- Half Window-Air Conduction1/RConn1 -- Door1/RConn1
  Thermal Mass InnerDoor1/LConn1 -- Door12/RConn1 -- Half Window-Air Conduction2/RConn1
  Half Wall-Air Conduction3/RConn1 -- 2-4/RConn1 -- Thermal Mass 2-4/LConn1
  Air-InnerWall IW2-4/RConn1 -- Half Wall-Air Conduction3/LConn1
  Air-InnerDoor Convection2/RConn1 -- Half Window-Air Conduction2/LConn1
  Air-InnerDoor Convection4/RConn1 -- Half Window-Air Conduction4/LConn1
  Air-InnerDoor Convection1/RConn1 -- Half Window-Air Conduction1/LConn1
  Air-InnerDoor Convection3/RConn1 -- Half Window-Air Conduction3/LConn1
  IW2-3/RConn1 -- Half Wall-Air Conduction2/LConn1
  Air-InnerDoor Convection5/RConn1 -- Half Window-Air Conduction5/LConn1
  IW2-1/RConn1 -- Half Wall-Air Conduction1/LConn1
  Air-InnerWall 2-12/RConn1 -- Half Wall-Air Conduction5/LConn1
  Air-InnerWall IW2-11/RConn1 -- Half Wall-Air Conduction4/LConn1
  Thermal Mass Flur2OG2/LConn1 -- Y-Flur2OG2/RConn1 -- Half Flur2OG2/RConn1
  Flur2OG2/RConn1 -- Half Flur2OG2/LConn1

== system Main_SpeedOptimisedVersionTannenweg/EG/Raum3 ==
  Tatm : Inport
  valve command : Inport  Port=2
  Controlled Temperature Source : fl_lib/Thermal/Thermal Sources/Controlled Temperature Source
  Flur3OG2 : fl_lib/Thermal/Thermal Elements/Convective Heat Transfer  thermal_type=foundation.enum.constant_variable.constant  area=15.87 m^2  heat_tr_coeff=8 W/m^2/K  min_heat_tr_coeff=1e-3 W/(K*m^2)  T_specify=off  T_priority=High  T=0 K  T_nominal_specify=off  T_nominal_value=1  T_nominal_unit=K  Q_specify=off  Q_priority=High  Q=0 J/s  Q_nominal_specify=off  Q_nominal_value=1  Q_nominal_unit=W
  Half Flur3OG2 : fl_lib/Thermal/Thermal Elements/Conductive Heat Transfer  thermal_type=foundation.enum.ConstantVariableTabulated.Constant  wall_geometry=foundation.enum.ConductionWallGeometry.Planar  area=15.87 m^2  thickness=.15 m  d_in=0.05 m  d_out=0.1 m  L=1 m  th_cond_min=10 W/(K*m)  th_cond=.32 W/m/K  th_cond_TLU=[413, 401, 392, 383, 371, 357, 342] W/(K*m)  temp_TLU=[200, 273, 400, 600, 800, 1000, 1200] K  T_specify=off  T_priority=High  T=0 K  T_nominal_specify=off  T_nominal_value=1  T_nominal_unit=K  Q_specify=off  Q_priority=High  Q=0 J/s  Q_nominal_specify=off  Q_nominal_value=1  Q_nominal_unit=W
  Half IT-Air1 : fl_lib/Thermal/Thermal Elements/Conductive Heat Transfer  thermal_type=foundation.enum.ConstantVariableTabulated.Constant  wall_geometry=foundation.enum.ConductionWallGeometry.Planar  area=1.8 m^2  thickness=.022 m  d_in=0.05 m  d_out=0.1 m  L=1 m  th_cond_min=10 W/(K*m)  th_cond=.13 W/m/K  th_cond_TLU=[413, 401, 392, 383, 371, 357, 342] W/(K*m)  temp_TLU=[200, 273, 400, 600, 800, 1000, 1200] K  T_specify=off  T_priority=High  T=0 K  T_nominal_specify=off  T_nominal_value=1  T_nominal_unit=K  Q_specify=off  Q_priority=High  Q=0 J/s  Q_nominal_specify=off  Q_nominal_value=1  Q_nominal_unit=W
  Half IT-Air2 : fl_lib/Thermal/Thermal Elements/Conductive Heat Transfer  thermal_type=foundation.enum.ConstantVariableTabulated.Constant  wall_geometry=foundation.enum.ConductionWallGeometry.Planar  area=8.4 m^2  thickness=.022 m  d_in=0.05 m  d_out=0.1 m  L=1 m  th_cond_min=10 W/(K*m)  th_cond=.13 W/m/K  th_cond_TLU=[413, 401, 392, 383, 371, 357, 342] W/(K*m)  temp_TLU=[200, 273, 400, 600, 800, 1000, 1200] K  T_specify=off  T_priority=High  T=0 K  T_nominal_specify=off  T_nominal_value=1  T_nominal_unit=K  Q_specify=off  Q_priority=High  Q=0 J/s  Q_nominal_specify=off  Q_nominal_value=1  Q_nominal_unit=W
  Half IW1-Air : fl_lib/Thermal/Thermal Elements/Conductive Heat Transfer  thermal_type=foundation.enum.ConstantVariableTabulated.Constant  wall_geometry=foundation.enum.ConductionWallGeometry.Planar  area=6.7 m^2  thickness=.16 m  d_in=0.05 m  d_out=0.1 m  L=1 m  th_cond_min=10 W/(K*m)  th_cond=.069 W/m/K  th_cond_TLU=[413, 401, 392, 383, 371, 357, 342] W/(K*m)  temp_TLU=[200, 273, 400, 600, 800, 1000, 1200] K  T_specify=off  T_priority=High  T=0 K  T_nominal_specify=off  T_nominal_value=1  T_nominal_unit=K  Q_specify=off  Q_priority=High  Q=0 J/s  Q_nominal_specify=off  Q_nominal_value=1  Q_nominal_unit=W
  Half IW1-Air1 : fl_lib/Thermal/Thermal Elements/Conductive Heat Transfer  thermal_type=foundation.enum.ConstantVariableTabulated.Constant  wall_geometry=foundation.enum.ConductionWallGeometry.Planar  area=8.5 m^2  thickness=.16 m  d_in=0.05 m  d_out=0.1 m  L=1 m  th_cond_min=10 W/(K*m)  th_cond=.069 W/m/K  th_cond_TLU=[413, 401, 392, 383, 371, 357, 342] W/(K*m)  temp_TLU=[200, 273, 400, 600, 800, 1000, 1200] K  T_specify=off  T_priority=High  T=0 K  T_nominal_specify=off  T_nominal_value=1  T_nominal_unit=K  Q_specify=off  Q_priority=High  Q=0 J/s  Q_nominal_specify=off  Q_nominal_value=1  Q_nominal_unit=W
  Heater : Subsystem
      settings: PortSchema="{\"entries\":[{\"content\":{\"sides\":[{\"content\":{\"connectorIds\":[\"In1\"]},\"type\":\"ConnectorPlacement.EquallySpacedRectSide\",\"uuid\":\"7b4379d5-fe86-4f5f-b347-17463247d5cb\"},{\"content\":{\"connectorIds\":[\"RConn1\"],\"side\":\"RIGHT\"},\"type\":\"ConnectorPlacement.EquallySpacedRectSide\",\"uuid\":\"add3919f-9a79-4726-aacf-5344366c736f\"},{\"content\":{\"connectorIds\":[\"LConn1\"],\"side\":\"TOP\"},\"type\":\"ConnectorPlacement.EquallySpacedRectSide\",\"uuid\":\"2be7b118-9114-410d-904a-4756a3068fbb\"},{\"content\":{\"connectorIds\":[\"RConn2\"],\"side\":\"BOTTOM\"},\"type\":\"ConnectorPlacement.EquallySpacedRectSide\",\"uuid\":\"3477f1e1-5c09-4719-a7a1-17d4fd79a7ad\"}]},\"type\":\"ConnectorPlacement.EquallySpacedConnector\",\"uuid\":\"01d92670-8519-469a-8463-0c3952b88216\"}],\"packageUris\":[\"http://schema.mathworks.com/mf0/Connector/R2020b\"],\"version\":\"1.0\"}"
  IT3 : fl_lib/Thermal/Thermal Elements/Convective Heat Transfer  thermal_type=foundation.enum.constant_variable.constant  area=1.8 m^2  heat_tr_coeff=8 W/m^2/K  min_heat_tr_coeff=1e-3 W/(K*m^2)  T_specify=off  T_priority=High  T=0 K  T_nominal_specify=off  T_nominal_value=1  T_nominal_unit=K  Q_specify=off  Q_priority=High  Q=0 J/s  Q_nominal_specify=off  Q_nominal_value=1  Q_nominal_unit=W
  IW3-12 : fl_lib/Thermal/Thermal Elements/Convective Heat Transfer  thermal_type=foundation.enum.constant_variable.constant  area=8.4 m^2  heat_tr_coeff=8 W/m^2/K  min_heat_tr_coeff=1e-3 W/(K*m^2)  T_specify=off  T_priority=High  T=0 K  T_nominal_specify=off  T_nominal_value=1  T_nominal_unit=K  Q_specify=off  Q_priority=High  Q=0 J/s  Q_nominal_specify=off  Q_nominal_value=1  Q_nominal_unit=W
  IW3-2 : fl_lib/Thermal/Thermal Elements/Convective Heat Transfer  thermal_type=foundation.enum.constant_variable.constant  area=6.7 m^2  heat_tr_coeff=8 W/m^2/K  min_heat_tr_coeff=1e-3 W/(K*m^2)  T_specify=off  T_priority=High  T=0 K  T_nominal_specify=off  T_nominal_value=1  T_nominal_unit=K  Q_specify=off  Q_priority=High  Q=0 J/s  Q_nominal_specify=off  Q_nominal_value=1  Q_nominal_unit=W
  IW3-4 : fl_lib/Thermal/Thermal Elements/Convective Heat Transfer  thermal_type=foundation.enum.constant_variable.constant  area=8.5 m^2  heat_tr_coeff=8 W/m^2/K  min_heat_tr_coeff=1e-3 W/(K*m^2)  T_specify=off  T_priority=High  T=0 K  T_nominal_specify=off  T_nominal_value=1  T_nominal_unit=K  Q_specify=off  Q_priority=High  Q=0 J/s  Q_nominal_specify=off  Q_nominal_value=1  Q_nominal_unit=W
  Simulink-PS Converter3 : nesl_utility/Simulink-PS Converter  PhysicalDomain=network_engine_domain  SubClassName=ps_input  LeftPortType=input  RightPortType=output  PseudoPeriodic=off  Frequencies=[]  NoiseDistribution=none  NoiseParameters=[]  Unit=degC  AffineConversion=on  FilteringAndDerivatives=zero  SimscapeFilterOrder=1  InputFilterTimeConstant=.001  UdotUserProvided=0
  Temp. Sensor : Subsystem
  Thermal Mass 3-12 : fl_lib/Thermal/Thermal Elements/Thermal Mass  mass_type=foundation.enum.constant_variable.constant  mass=8.4*.15*547 kg  sp_heat=1600 J/kg/K  mass_min=1e-6 kg  num_ports=foundation.enum.numPorts2.one  m_specify=off  m_priority=High  m=1 kg  m_nominal_specify=off  m_nominal_value=1  m_nominal_unit=kg  T_specify=on  T_priority=High  T=Ti degC  T_nominal_specify=off  T_nominal_value=1  T_nominal_unit=K  Q_specify=off  Q_priority=None  Q=0 W  Q_nominal_specify=off  Q_nominal_value=1  Q_nominal_unit=W
  Thermal Mass Air : fl_lib/Thermal/Thermal Elements/Thermal Mass  mass_type=foundation.enum.constant_variable.constant  mass=48.7 kg  sp_heat=1005 J/kg/K  mass_min=1e-6 kg  num_ports=foundation.enum.numPorts2.one  m_specify=off  m_priority=High  m=1 kg  m_nominal_specify=off  m_nominal_value=1  m_nominal_unit=kg  T_specify=on  T_priority=High  T=Ti degC  T_nominal_specify=off  T_nominal_value=1  T_nominal_unit=K  Q_specify=off  Q_priority=None  Q=0 W  Q_nominal_specify=off  Q_nominal_value=1  Q_nominal_unit=W
  Thermal Mass Door3 : fl_lib/Thermal/Thermal Elements/Thermal Mass  mass_type=foundation.enum.constant_variable.constant  mass=36 kg  sp_heat=1600 J/kg/K  mass_min=1e-6 kg  num_ports=foundation.enum.numPorts2.one  m_specify=off  m_priority=High  m=1 kg  m_nominal_specify=off  m_nominal_value=1  m_nominal_unit=kg  T_specify=on  T_priority=High  T=Ti degC  T_nominal_specify=off  T_nominal_value=1  T_nominal_unit=K  Q_specify=off  Q_priority=None  Q=0 W  Q_nominal_specify=off  Q_nominal_value=1  Q_nominal_unit=W
  Thermal Mass Flur3OG2 : fl_lib/Thermal/Thermal Elements/Thermal Mass  mass_type=foundation.enum.constant_variable.constant  mass=4473 kg  sp_heat=889 J/kg/K  mass_min=1e-6 kg  num_ports=foundation.enum.numPorts2.one  m_specify=off  m_priority=High  m=1 kg  m_nominal_specify=off  m_nominal_value=1  m_nominal_unit=kg  T_specify=on  T_priority=High  T=Ti degC  T_nominal_specify=off  T_nominal_value=1  T_nominal_unit=K  Q_specify=off  Q_priority=None  Q=0 W  Q_nominal_specify=off  Q_nominal_value=1  Q_nominal_unit=W
  Thermal Mass IW3-2 : fl_lib/Thermal/Thermal Elements/Thermal Mass  mass_type=foundation.enum.constant_variable.constant  mass=6.7*.15*547 kg  sp_heat=1600 J/kg/K  mass_min=1e-6 kg  num_ports=foundation.enum.numPorts2.one  m_specify=off  m_priority=High  m=1 kg  m_nominal_specify=off  m_nominal_value=1  m_nominal_unit=kg  T_specify=on  T_priority=High  T=Ti degC  T_nominal_specify=off  T_nominal_value=1  T_nominal_unit=K  Q_specify=off  Q_priority=None  Q=0 W  Q_nominal_specify=off  Q_nominal_value=1  Q_nominal_unit=W
  Thermal Mass IW3-4 : fl_lib/Thermal/Thermal Elements/Thermal Mass  mass_type=foundation.enum.constant_variable.constant  mass=8.5*.15*547 kg  sp_heat=1600 J/kg/K  mass_min=1e-6 kg  num_ports=foundation.enum.numPorts2.one  m_specify=off  m_priority=High  m=1 kg  m_nominal_specify=off  m_nominal_value=1  m_nominal_unit=kg  T_specify=on  T_priority=High  T=Ti degC  T_nominal_specify=off  T_nominal_value=1  T_nominal_unit=K  Q_specify=off  Q_priority=None  Q=0 W  Q_nominal_specify=off  Q_nominal_value=1  Q_nominal_unit=W
  Thermal Reference1 : fl_lib/Thermal/Thermal Elements/Thermal Reference
  X-Atm : Subsystem
  Hot Water In1 : PMIOPort  Side=Left
  3-12 : PMIOPort  Port=2  Side=Left
  Door3 : PMIOPort  Port=3  Side=Left
  Y-Flur3OG2 : PMIOPort  Port=4  Side=Left
  3-2 : PMIOPort  Port=5  Side=Right
  3-4 : PMIOPort  Port=6  Side=Right
  Hot Water Out1 : PMIOPort  Port=7  Side=Right
  Troom : Outport
  wires:
  Temp. Sensor/1(T) -> Troom/1
  Tatm/1 -> Simulink-PS Converter3/1
  valve command/1 -> Heater/1(valve command)
  connections:
  IW3-2/RConn1 -- Half IW1-Air/LConn1
  3-2/RConn1 -- Thermal Mass IW3-2/LConn1 -- Half IW1-Air/RConn1
  Thermal Reference1/LConn1 -- Controlled Temperature Source/RConn2
  Controlled Temperature Source/RConn1 -- Simulink-PS Converter3/RConn1
  Thermal Mass Air/LConn1 -- Flur3OG2/LConn1 -- IT3/LConn1 -- IW3-12/LConn1 -- IW3-4/LConn1 -- IW3-2/LConn1 -- Heater/RConn1 -- Temp. Sensor/LConn1 -- X-Atm/LConn1
  X-Atm/RConn1 -- Controlled Temperature Source/LConn1
  Hot Water In1/RConn1 -- Heater/LConn1
  Heater/RConn2 -- Hot Water Out1/RConn1
  Thermal Mass IW3-4/LConn1 -- Half IW1-Air1/RConn1 -- 3-4/RConn1
  IW3-4/RConn1 -- Half IW1-Air1/LConn1
  Half IT-Air2/RConn1 -- Thermal Mass 3-12/LConn1 -- 3-12/RConn1
  IW3-12/RConn1 -- Half IT-Air2/LConn1
  Thermal Mass Door3/LConn1 -- Door3/RConn1 -- Half IT-Air1/RConn1
  IT3/RConn1 -- Half IT-Air1/LConn1
  Thermal Mass Flur3OG2/LConn1 -- Y-Flur3OG2/RConn1 -- Half Flur3OG2/RConn1
  Flur3OG2/RConn1 -- Half Flur3OG2/LConn1
